simulink model "case3_primary_AGC_GFM"  (R2024b)
settings: Solver=ode15s  StartTime=0.0  StopTime=t_stop  MaxStep=0.01  RelTol=1e-6
model workspace (MATLAB code in the model file):
  | %% TWO-MACHINE SYSTEM  -  model data
  | % Case 3 - primary + secondary control (AGC) + GFM
  | % Rodriguez-Amenedo & Arnaltes Gomez, IEEE Access 9 (2021), Fig. 14.
  | % Per unit on Sbase = 100 MVA, f0 = 50 Hz, phasor (RMS) model.
  | % This code is stored in the model (Model Explorer > Model Workspace) and
  | % runs automatically when the model is opened. Edit the values here and
  | % click "Reinitialize from Source" to apply them.
  | 
  | %% Disturbance and simulation time
  | dP_L2_MW = -100;     % load step at bus 2 [MW] (paper: -100 MW, load rejection)
  | t_step   = 1;        % time of the load step [s]
  | t_stop   = 150;      % simulation time [s] (the slow AGC settles in about 125 s)
  | 
  | %% System base
  | Sbase = 100;         % [MVA]
  | f0    = 50;          % [Hz]
  | ws    = 2*pi*f0;     % [rad/s]
  | 
  | %% Network reactances [pu on 100 MVA]
  | x_T1 = 0.01;         % transformer SG1, bus 1-2
  | x_T5 = 0.01;         % transformer GFM, bus 5-2 (bus 5 = GFM connection point)
  | x_T2 = 0.003;        % transformer SG2, bus 3-4
  | x_L  = 0.2/2;        % two parallel 0.2 pu tie-lines, bus 2-3
  | 
  | %% Operating point (paper Table 2)
  | P_SG1 = 1350;                            % SG1 dispatch [MW]
  | P_L2  = 1250;  P_L3  = 4000;             % loads [MW], unity power factor
  | V1    = 1.0;   V4    = 1.0;              % [pu]; bus 4 (SG2) is the slack
  | P_GFM = 0;     Q_GFM = 0;                % GFM dispatch [MW], [MVAr]
  | 
  | %% Synchronous generators - model 0.0, classical (own rating)
  | % Constant emf E' behind the transient reactance x'd; no rotor circuits,
  | % no exciter.
  | S1  = 1500;  S2 = 4000;      % ratings [MVA]
  | H   = 6.3;                   % inertia constant [s]
  | D   = 0;                     % rotor damping [pu torque / pu speed, own base] (paper)
  | D_load = 1;                  % load damping [pu load change / pu frequency change,
  |                              % load base]: typical 1-2 (Kundur 1994, Sec. 11.1.3),
  |                              % lower end used. The paper's loads have no frequency
  |                              % dependence; the load damping is lumped into the swing
  |                              % equations as in the standard LFC model, 1/(2Hs + D).
  | D1  = D + D_load*P_L2/S1;    % total damping SG1 [pu, own base] (Area-1 load, bus 2)
  | D2  = D + D_load*P_L3/S2;    % total damping SG2 [pu, own base] (Area-2 load, bus 3)
  | xdp = 0.34;                  % transient reactance x'd [pu]
  | 
  | %% Governor and turbine - IEEEG1 (paper Table 7), primary control
  | K   = 20;                    % governor gain 1/R (5 % droop)
  | T3  = 0.1;                   % servo time constant [s]
  | Uo  = 0.5;   Uc = -0.5;      % valve rate limits [pu/s]
  | Pmax = 1;    Pmin = 0;       % valve position limits [pu]
  | T4  = 0.3;   T5 = 7;   T6 = 0.6;      % steam chest, reheater, crossover [s]
  | K1  = 0.3;   K3 = 0.3; K5 = 0.4;      % HP, IP, LP power fractions
  | 
  | kS1 = S1/Sbase;   xd1 = xdp/kS1;      % x'd of SG1 on 100 MVA
  | kS2 = S2/Sbase;   xd2 = xdp/kS2;      % x'd of SG2 on 100 MVA
  | 
  | %% Secondary control - tie-line bias AGC
  | % Area 1 = SG1 (+ GFM), Area 2 = SG2. Bias B = area frequency response
  | % (set in the AGC block). Ki: integral gain [pu set-point / pu ACE / s].
  | Ki = 0.02;     % low gain: AGC about 6-7 times slower than primary control
  | 
  | %% Grid-forming converter (own rating)
  | Sg  = 1500;                  % rating [MVA]
  | kSg = Sg/Sbase;
  | xg  = 0.15/kSg;              % coupling reactance on 100 MVA
  | Rg  = 0.05;                  % P-f droop [pu]
  | Kw  = 3;    Tw = 1;          % POD-P washout gain [pu] and time constant [s]
  | pod_on = 0;                  % 0 = pure P-f droop (POD-P washout loop off), 1 = droop + POD-P
  | Tf  = 0.02;                  % bus-frequency measurement filter [s]
  | 
  | %% Bus admittance matrix (buses 1..5)
  | Ybus     = zeros(5);
  | branches = [1 2 x_T1; 5 2 x_T5; 3 4 x_T2; 2 3 x_L];   % [from to x]
  | for k = 1:size(branches, 1)
  |     i = branches(k,1);  j = branches(k,2);  y = 1/(1i*branches(k,3));
  |     Ybus([i j], [i j]) = Ybus([i j], [i j]) + [y -y; -y y];
  | end
  | 
  | %% Load flow (Newton-Raphson)
  | % Unknowns z = [th1 th2 th3 th5 V2 V3 V5]; bus 1 PV, buses 2,3,5 PQ.
  | Vbus  = @(z) [V1*exp(1i*z(1)); z(5)*exp(1i*z(2)); z(6)*exp(1i*z(3)); V4; z(7)*exp(1i*z(4))];
  | Sinj  = @(V) V .* conj(Ybus*V);
  | PQ    = @(S) [real(S([1 2 3 5])); imag(S([2 3 5]))];
  | spec  = [P_SG1; -P_L2; -P_L3; P_GFM; 0; 0; Q_GFM] / Sbase;
  | mis   = @(z) PQ(Sinj(Vbus(z))) - spec;
  | 
  | z = [0; 0; 0; 0; 1; 1; 1];
  | for it = 1:20
  |     J = zeros(7);
  |     for k = 1:7
  |         dz = zeros(7,1);  dz(k) = 1e-7;
  |         J(:,k) = (mis(z + dz) - mis(z)) / 1e-7;
  |     end
  |     z = z - J \ mis(z);
  | end
  | if norm(mis(z)) > 1e-9
  |     error('Load flow did not converge (mismatch %.1e pu).', norm(mis(z)));
  | end
  | V0 = Vbus(z);                % bus voltages [pu]
  | S0 = Sinj(V0);               % bus injections [pu]
  | 
  | %% Initial values of the synchronous generators: E' = V + j x'd I
  | E1 = V0(1) + 1i*xd1*conj(S0(1)/V0(1));
  | E2 = V0(4) + 1i*xd2*conj(S0(4)/V0(4));
  | E1_mag = abs(E1);   delta1_0 = angle(E1);      % |E'| is held fixed
  | E2_mag = abs(E2);   delta2_0 = angle(E2);
  | Pm1_0  = real(S0(1)) / kS1;                  % governor set-points [pu own]
  | Pm2_0  = real(S0(4)) / kS2;
  | Ptie_0 = real(V0(2) * conj((V0(2) - V0(3)) / (1i*x_L)));   % scheduled tie flow [pu]
  | 
  | %% Initial values of the GFM: Eg = V + j xg I  (|Eg| is held fixed)
  | Eg = V0(5) + 1i*xg*conj(S0(5)/V0(5));
  | Eg_mag   = abs(Eg);   deltag_0 = angle(Eg);
  | Pg_ref   = real(S0(5)) / kSg;                % GFM power reference [pu own]
  | theta5_0 = angle(V0(5));
  | 
  | %% Network impedance matrices (ZI loads, as in the paper)
  | % Loads are ZI loads: the active power is a constant current in phase with
  | % the bus voltage, I_L = I_L,mag * V/|V| (so P_L is proportional to |V|);
  | % the reactive power is a constant impedance (zero here: unity power factor).
  | % The SG transient reactances x'd are added at buses 1 and 4,
  | % the GFM reactance xg at bus 5 (Norton form like the SGs).
  | % Network block: V = Zn*J - ZnL*I_L (J: Norton currents of the sources).
  | yQ      = zeros(5,1);
  | yQ(2:3) = 1i*imag(conj(-S0(2:3)) ./ abs(V0(2:3)).^2);   % constant-Z reactive part
  | Yaug    = Ybus + diag(yQ);
  | Yaug(1,1) = Yaug(1,1) + 1/(1i*xd1);
  | Yaug(4,4) = Yaug(4,4) + 1/(1i*xd2);
  | Yaug(5,5) = Yaug(5,5) + 1/(1i*xg);     % GFM reactance, Norton form like the SGs
  | Z   = inv(Yaug);
  | Zn  = Z(:, [1 4 5]);       % columns of the source (Norton) injections
  | ZnL = Z(:, [2 3]);       % columns of the load buses 2 and 3
  | 
  | % Constant-current magnitudes [pu, 100 MVA]; the load step changes the
  | % current at bus 2 by dP_L2 at nominal voltage
  | IL_pre  = real(-S0(2:3)) ./ abs(V0(2:3));
  | IL_post = IL_pre + [dP_L2_MW/Sbase/abs(V0(2)); 0];
  | 
  | % Angle of the load currents: follows the bus-voltage angle (measured
  | % relative to the SG1 rotor, so it is continuous) through a fast lag that
  | % breaks the algebraic loop through the load buses (numerical only)
  | T_L      = 1e-4;                                         % [s]
  | thetaL_0 = delta1_0 + angle(V0(2:3) * exp(-1i*delta1_0));   % [rad]
  | 
  | % Check: the network must reproduce the load flow at t = 0
  | I0  = [E1/(1i*xd1); E2/(1i*xd2); Eg/(1i*xg)];
  | IL0 = IL_pre .* V0(2:3) ./ abs(V0(2:3));
  | if max(abs(Zn*I0 - ZnL*IL0 - V0)) > 1e-9
  |     error('Network initialization does not match the load flow.');
  | end
  | clear i j k y it dz J z I0 IL0 Z Yaug yQ branches Vbus Sinj PQ spec mis E1 E2
  | clear Eg
Description:
  | Case 3 - primary + secondary control (AGC) + GFM. Two-machine load-frequency model (SG model 0.0, classical). All data in the Model Workspace; press Run.
settings Model: Creator=Hussain  LastModifiedBy=Hussain
settings DataIOCC: SaveOutput=off
settings DebuggingCC: AlgebraicLoopMsg=error

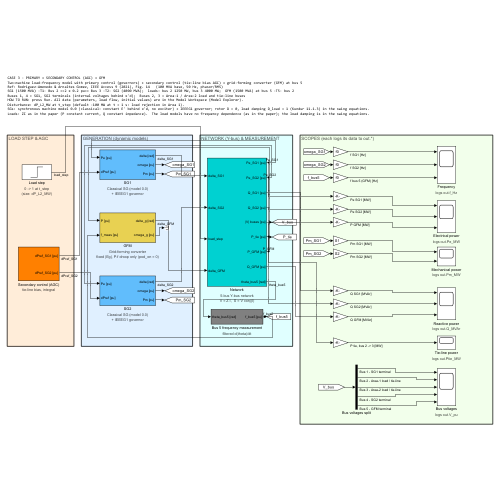
[thumbnail: Simulink's stored preview of the top-level diagram]
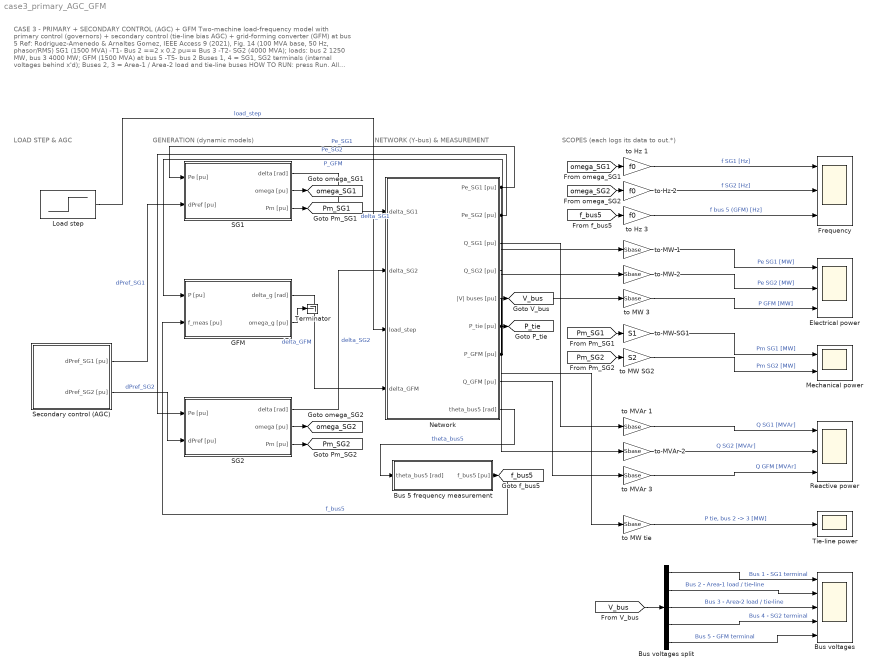
== system case3_primary_AGC_GFM ==
  note: LOAD STEP & AGC
  note: GENERATION (dynamic models)
  note: NETWORK (Y-bus) & MEASUREMENT
  note: SCOPES (each logs its data to out.*)
  note: CASE 3 - PRIMARY + SECONDARY CONTROL (AGC) + GFM
      | Two-machine load-frequency model with primary control (governors) + secondary control (tie-line bias AGC) + grid-forming converter (GFM) at bus 5
      | Ref: Rodriguez-Amenedo & Arnaltes Gomez, IEEE Access 9 (2021), Fig. 14   (100 MVA base, 50 Hz, phasor/RMS)
      | SG1 (1500 MVA) -T1- Bus 2 ==2 x 0.2 pu== Bus 3 -T2- SG2 (4000 MVA);  loads: bus 2 1250 MW, bus 3 4000 MW;  GFM (1500 MVA) at bus 5 -T5- bus 2
      | Buses 1, 4 = SG1, SG2 terminals (internal voltages behind x'd);  Buses 2, 3 = Area-1 / Area-2 load and tie-line buses
      | HOW TO RUN: press Run. All data (parameters, load flow, initial values) are in the Model Workspace (Model Explorer).
      | Disturbance: dP_L2_MW at t_step (default -100 MW at t = 1 s: load rejection in Area 1).
      | SGs: synchronous machine model 0.0 (classical: constant E' behind x'd, no exciter) + IEEEG1 governor; rotor D = 0, load damping D_load = 1 (Kundur 11.1.3) in the swing equations.
      | Loads: ZI as in the paper (P constant current, Q constant impedance).  The load models have no frequency dependence (as in the paper); the load damping is in the swing equations.
  Bus 5 frequency measurement : Subsystem
      settings: AttributesFormatString=filtered d(theta)/dt
  Bus voltages : Scope  NumInputPorts=5
      settings: AttributesFormatString=logs out.V_pu
  Bus voltages split : Demux  Outputs=5
  Electrical power : Scope  NumInputPorts=3
      settings: AttributesFormatString=logs out.Pe_MW
  Frequency : Scope  NumInputPorts=3
      settings: AttributesFormatString=logs out.f_Hz
  GFM : Subsystem
      settings: AttributesFormatString=Grid-forming converter\nfixed |Eg|, P-f droop only (pod_on = 0)
  Load step : Step  Time=t_step  SampleTime=0
      settings: AttributesFormatString=0 -> 1 at t_step\n(size: dP_L2_MW)
  Mechanical power : Scope  NumInputPorts=2
      settings: AttributesFormatString=logs out.Pm_MW
  Network : Subsystem
      settings: AttributesFormatString="5-bus Y-bus network\\nV = Z I,  S = V conj(I)"
  Reactive power : Scope  NumInputPorts=3
      settings: AttributesFormatString=logs out.Q_MVAr
  SG1 : Subsystem
      settings: AttributesFormatString=Classical SG (model 0.0)\n+ IEEEG1 governor
  SG2 : Subsystem
      settings: AttributesFormatString=Classical SG (model 0.0)\n+ IEEEG1 governor
  Secondary control (AGC) : Subsystem
      settings: AttributesFormatString=tie-line bias, integral
  Terminator : Terminator
  Tie-line power : Scope
      settings: AttributesFormatString=logs out.Ptie_MW
  to Hz 1 : Gain  Gain=f0
  to Hz 2 : Gain  Gain=f0
  to Hz 3 : Gain  Gain=f0
  to MVAr 1 : Gain  Gain=Sbase
  to MVAr 2 : Gain  Gain=Sbase
  to MVAr 3 : Gain  Gain=Sbase
  to MW 1 : Gain  Gain=Sbase
  to MW 2 : Gain  Gain=Sbase
  to MW 3 : Gain  Gain=Sbase
  to MW SG1 : Gain  Gain=S1
  to MW SG2 : Gain  Gain=S2
  to MW tie : Gain  Gain=Sbase
  tag scope: P_tie=global, Pm_SG1=global, Pm_SG2=global, V_bus=global, f_bus5=global, omega_SG1=global, omega_SG2=global
  wires:
  Secondary control (AGC)/1(dPref_SG1 [pu]) -> SG1/2(dPref [pu])  "dPref_SG1"
  Secondary control (AGC)/2(dPref_SG2 [pu]) -> SG2/2(dPref [pu])  "dPref_SG2"
  SG1/1(delta [rad]) -> Network/1(delta_SG1)  "delta_SG1"
  SG2/1(delta [rad]) -> Network/2(delta_SG2)  "delta_SG2"
  Load step/1 -> Network/3(load_step)  "load_step"
  Network/1(Pe_SG1 [pu]) -> SG1/1(Pe [pu]), to MW 1/1  "Pe_SG1"
  Network/2(Pe_SG2 [pu]) -> SG2/1(Pe [pu]), to MW 2/1  "Pe_SG2"
  SG1/2(omega [pu]) -> [omega_SG1]
  SG1/3(Pm [pu]) -> [Pm_SG1]
  SG2/2(omega [pu]) -> [omega_SG2]
  SG2/3(Pm [pu]) -> [Pm_SG2]
  Network/6(P_tie [pu]) -> [P_tie], to MW tie/1
  GFM/1(delta_g [rad]) -> Network/4(delta_GFM)  "delta_GFM"
  Network/7(P_GFM [pu]) -> GFM/1(P [pu]), to MW 3/1  "P_GFM"
  Network/9(theta_bus5 [rad]) -> Bus 5 frequency measurement/1(theta_bus5 [rad])  "theta_bus5"
  Bus 5 frequency measurement/1(f_bus5 [pu]) -> GFM/2(f_meas [pu]), [f_bus5]  "f_bus5"
  GFM/2(omega_g [pu]) -> Terminator/1
  [omega_SG1] -> to Hz 1/1
  [omega_SG2] -> to Hz 2/1
  [f_bus5] -> to Hz 3/1
  to Hz 1/1 -> Frequency/1  "f SG1 [Hz]"
  to Hz 2/1 -> Frequency/2  "f SG2 [Hz]"
  to Hz 3/1 -> Frequency/3  "f bus 5 (GFM) [Hz]"
  to MW 1/1 -> Electrical power/1  "Pe SG1 [MW]"
  to MW 2/1 -> Electrical power/2  "Pe SG2 [MW]"
  to MW 3/1 -> Electrical power/3  "P GFM [MW]"
  [Pm_SG1] -> to MW SG1/1
  [Pm_SG2] -> to MW SG2/1
  to MW SG1/1 -> Mechanical power/1  "Pm SG1 [MW]"
  to MW SG2/1 -> Mechanical power/2  "Pm SG2 [MW]"
  Network/3(Q_SG1 [pu]) -> to MVAr 1/1
  Network/4(Q_SG2 [pu]) -> to MVAr 2/1
  Network/8(Q_GFM [pu]) -> to MVAr 3/1
  to MVAr 1/1 -> Reactive power/1  "Q SG1 [MVAr]"
  to MVAr 2/1 -> Reactive power/2  "Q SG2 [MVAr]"
  to MVAr 3/1 -> Reactive power/3  "Q GFM [MVAr]"
  to MW tie/1 -> Tie-line power/1  "P tie, bus 2 -> 3 [MW]"
  Network/5(|V| buses [pu]) -> [V_bus]
  [V_bus] -> Bus voltages split/1
  Bus voltages split/1 -> Bus voltages/1  "Bus 1 - SG1 terminal"
  Bus voltages split/2 -> Bus voltages/2  "Bus 2 - Area-1 load / tie-line"
  Bus voltages split/3 -> Bus voltages/3  "Bus 3 - Area-2 load / tie-line"
  Bus voltages split/4 -> Bus voltages/4  "Bus 4 - SG2 terminal"
  Bus voltages split/5 -> Bus voltages/5  "Bus 5 - GFM terminal"

== system case3_primary_AGC_GFM/Bus 5 frequency measurement ==
  note: BUS FREQUENCY MEASUREMENT (bus 5, GFM terminal)
      | Tf dx/dt = theta - x,    f = 1 + (theta - x) / (Tf omega_s)   [pu]
      | A first-order filtered derivative of the bus voltage angle.
  theta_bus5 [rad] : Inport
  Angle error : Sum  Inputs=+-
  Bus frequency : Sum
  Filtered angle : Integrator  InitialCondition=theta5_0
  Nominal 1 pu : Constant
  One over Tf : Gain  Gain=1/Tf
  to pu frequency : Gain  Gain=1/ws
  f_bus5 [pu] : Outport
  wires:
  One over Tf/1 -> Filtered angle/1, to pu frequency/1  "d(theta)/dt"
  Bus frequency/1 -> f_bus5 [pu]/1  "f_bus5"
  to pu frequency/1 -> Bus frequency/2
  Nominal 1 pu/1 -> Bus frequency/1
  Angle error/1 -> One over Tf/1
  theta_bus5 [rad]/1 -> Angle error/1
  Filtered angle/1 -> Angle error/2

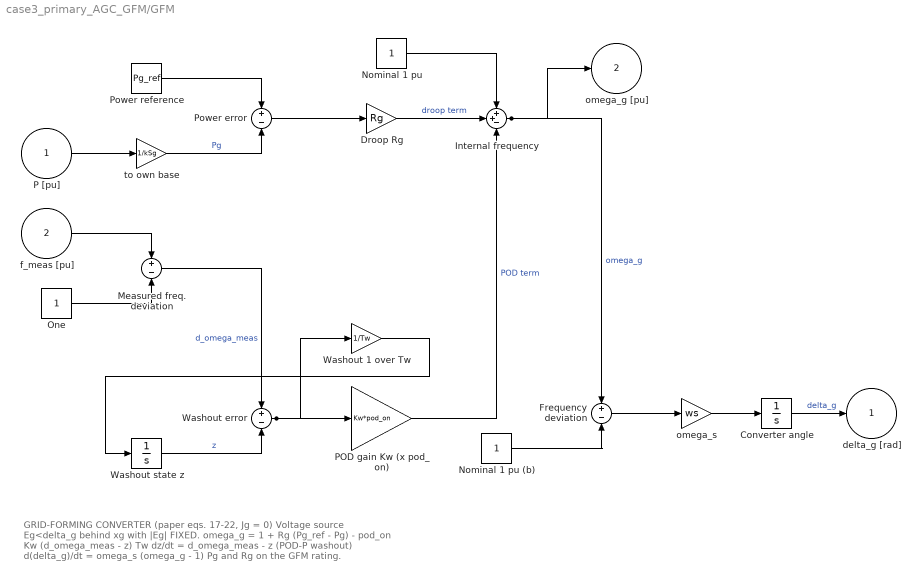
== system case3_primary_AGC_GFM/GFM ==
  note: GRID-FORMING CONVERTER (paper eqs. 17-22, Jg = 0)
      | Voltage source Eg<delta_g behind xg with |Eg| FIXED.
      | omega_g = 1 + Rg (Pg_ref - Pg) - pod_on Kw (d_omega_meas - z)
      | Tw dz/dt = d_omega_meas - z          (POD-P washout)
      | d(delta_g)/dt = omega_s (omega_g - 1)
      | Pg and Rg on the GFM rating.
  P [pu] : Inport
  f_meas [pu] : Inport  Port=2
  Converter angle : Integrator  InitialCondition=deltag_0
  Droop Rg : Gain  Gain=Rg
  Frequency deviation : Sum  Inputs=+-
  Internal frequency : Sum  Inputs=++-
  Measured freq. deviation : Sum  Inputs=+-
  Nominal 1 pu : Constant
  Nominal 1 pu (b) : Constant
  One : Constant
  POD gain Kw (x pod_on) : Gain  Gain=Kw*pod_on
  Power error : Sum  Inputs=+-
  Power reference : Constant  Value=Pg_ref
  Washout 1 over Tw : Gain  Gain=1/Tw
  Washout error : Sum  Inputs=+-
  Washout state z : Integrator
  omega_s : Gain  Gain=ws
  to own base : Gain  Gain=1/kSg
  delta_g [rad] : Outport
  omega_g [pu] : Outport  Port=2
  wires:
  P [pu]/1 -> to own base/1
  f_meas [pu]/1 -> Measured freq. deviation/1
  Converter angle/1 -> delta_g [rad]/1  "delta_g"
  Measured freq. deviation/1 -> Washout error/1  "d_omega_meas"
  One/1 -> Measured freq. deviation/2
  Power error/1 -> Droop Rg/1
  Power reference/1 -> Power error/1
  Washout state z/1 -> Washout error/2  "z"
  to own base/1 -> Power error/2  "Pg"
  Washout error/1 -> POD gain Kw (x pod_on)/1, Washout 1 over Tw/1
  Nominal 1 pu/1 -> Internal frequency/1
  Frequency deviation/1 -> omega_s/1
  Droop Rg/1 -> Internal frequency/2  "droop term"
  Washout 1 over Tw/1 -> Washout state z/1
  POD gain Kw (x pod_on)/1 -> Internal frequency/3  "POD term"
  Internal frequency/1 -> Frequency deviation/1, omega_g [pu]/1  "omega_g"
  Nominal 1 pu (b)/1 -> Frequency deviation/2
  omega_s/1 -> Converter angle/1

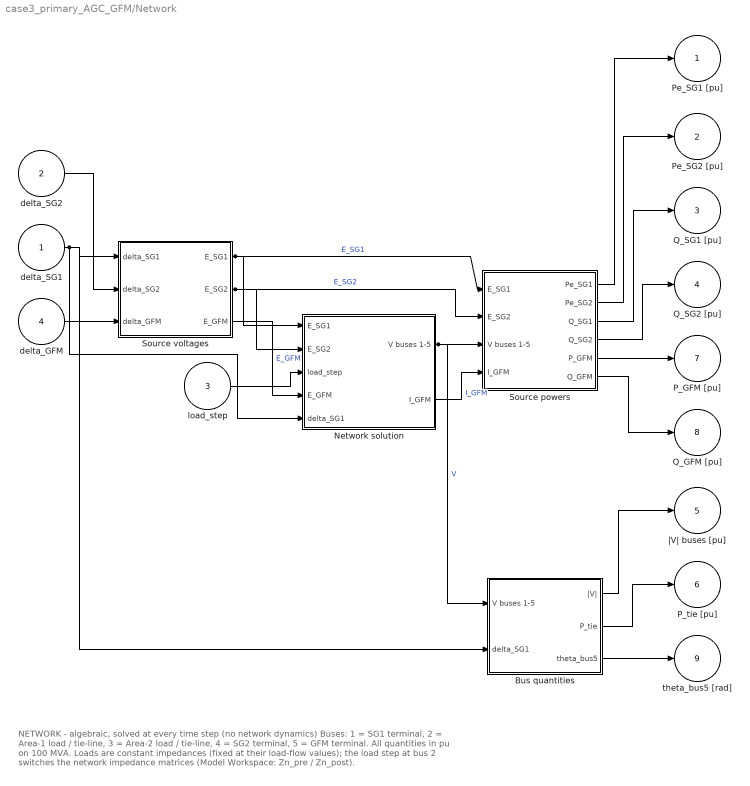
== system case3_primary_AGC_GFM/Network ==
  note: NETWORK - algebraic, solved at every time step (no network dynamics)
      | Buses: 1 = SG1 terminal, 2 = Area-1 load / tie-line, 3 = Area-2 load / tie-line,
      |        4 = SG2 terminal, 5 = GFM terminal.  All quantities in pu on 100 MVA.
      | Loads are constant impedances (fixed at their load-flow values); the load step at
      | bus 2 switches the network impedance matrices (Model Workspace: Zn_pre / Zn_post).
  delta_SG1 : Inport
  delta_SG2 : Inport  Port=2
  load_step : Inport  Port=3
  delta_GFM : Inport  Port=4
  Bus quantities : Subsystem
      settings: AttributesFormatString=|V|, tie-line flow, bus-5 angle
  Network solution : Subsystem
      settings: AttributesFormatString=V = Zn [J_SG1; J_SG2; J_GFM]
  Source powers : Subsystem
      settings: AttributesFormatString=S = V_terminal conj(I)
  Source voltages : Subsystem
      settings: AttributesFormatString=E = |E| at angle delta
  Pe_SG1 [pu] : Outport
  Pe_SG2 [pu] : Outport  Port=2
  Q_SG1 [pu] : Outport  Port=3
  Q_SG2 [pu] : Outport  Port=4
  |V| buses [pu] : Outport  Port=5
  P_tie [pu] : Outport  Port=6
  P_GFM [pu] : Outport  Port=7
  Q_GFM [pu] : Outport  Port=8
  theta_bus5 [rad] : Outport  Port=9
  wires:
  delta_SG2/1 -> Source voltages/2(delta_SG2)
  load_step/1 -> Network solution/3(load_step)
  delta_SG1/1 -> Bus quantities/2(delta_SG1), Source voltages/1(delta_SG1), Network solution/5(delta_SG1)
  Network solution/1(V buses 1-5) -> Source powers/3(V buses 1-5), Bus quantities/1(V buses 1-5)  "V"
  delta_GFM/1 -> Source voltages/3(delta_GFM)
  Source voltages/1(E_SG1) -> Source powers/1(E_SG1), Network solution/1(E_SG1)  "E_SG1"
  Source voltages/3(E_GFM) -> Network solution/4(E_GFM)  "E_GFM"
  Source voltages/2(E_SG2) -> Source powers/2(E_SG2), Network solution/2(E_SG2)  "E_SG2"
  Network solution/2(I_GFM) -> Source powers/4(I_GFM)  "I_GFM"
  Source powers/1(Pe_SG1) -> Pe_SG1 [pu]/1
  Source powers/2(Pe_SG2) -> Pe_SG2 [pu]/1
  Source powers/3(Q_SG1) -> Q_SG1 [pu]/1
  Source powers/4(Q_SG2) -> Q_SG2 [pu]/1
  Source powers/5(P_GFM) -> P_GFM [pu]/1
  Source powers/6(Q_GFM) -> Q_GFM [pu]/1
  Bus quantities/1(|V|) -> |V| buses [pu]/1
  Bus quantities/2(P_tie) -> P_tie [pu]/1
  Bus quantities/3(theta_bus5) -> theta_bus5 [rad]/1

== system case3_primary_AGC_GFM/SG1 ==
  note: SG1 - SYNCHRONOUS GENERATOR, MODEL 0.0 (classical)
      | Constant emf E'1 behind x'd (no rotor circuits, no exciter). The network returns Pe;
      | the swing equation gives speed and rotor angle; governor + turbine set Pm.
  Pe [pu] : Inport
  dPref [pu] : Inport  Port=2
  Governor (IEEEG1) : Subsystem
  Swing equation : Subsystem
  Turbine (reheat) : Subsystem
  delta [rad] : Outport
  omega [pu] : Outport  Port=2
  Pm [pu] : Outport  Port=3
  wires:
  Turbine (reheat)/1(Pm [pu]) -> Swing equation/1(Pm [pu own]), Pm [pu]/1  "Pm"
  Pe [pu]/1 -> Swing equation/2(Pe [pu 100 MVA])  "Pe"
  Swing equation/1(delta [rad]) -> delta [rad]/1  "delta"
  dPref [pu]/1 -> Governor (IEEEG1)/2(dPref (AGC) [pu])  "dPref"
  Governor (IEEEG1)/1(valve gv [pu]) -> Turbine (reheat)/1(valve gv [pu])  "gv"
  Swing equation/2(omega [pu]) -> Governor (IEEEG1)/1(omega [pu]), omega [pu]/1  "omega"

== system case3_primary_AGC_GFM/SG2 ==
  note: SG2 - SYNCHRONOUS GENERATOR, MODEL 0.0 (classical)
      | Constant emf E'2 behind x'd (no rotor circuits, no exciter). The network returns Pe;
      | the swing equation gives speed and rotor angle; governor + turbine set Pm.
  Pe [pu] : Inport
  dPref [pu] : Inport  Port=2
  Governor (IEEEG1) : Subsystem
  Swing equation : Subsystem
  Turbine (reheat) : Subsystem
  delta [rad] : Outport
  omega [pu] : Outport  Port=2
  Pm [pu] : Outport  Port=3
  wires:
  Turbine (reheat)/1(Pm [pu]) -> Swing equation/1(Pm [pu own]), Pm [pu]/1  "Pm"
  Pe [pu]/1 -> Swing equation/2(Pe [pu 100 MVA])  "Pe"
  dPref [pu]/1 -> Governor (IEEEG1)/2(dPref (AGC) [pu])  "dPref"
  Swing equation/1(delta [rad]) -> delta [rad]/1  "delta"
  Governor (IEEEG1)/1(valve gv [pu]) -> Turbine (reheat)/1(valve gv [pu])  "gv"
  Swing equation/2(omega [pu]) -> Governor (IEEEG1)/1(omega [pu]), omega [pu]/1  "omega"

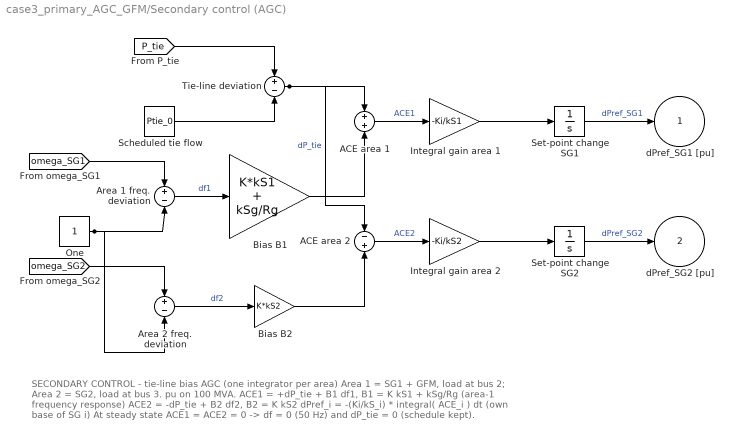
== system case3_primary_AGC_GFM/Secondary control (AGC) ==
  note: SECONDARY CONTROL - tie-line bias AGC (one integrator per area)
      | Area 1 = SG1 + GFM, load at bus 2;  Area 2 = SG2, load at bus 3.  pu on 100 MVA.
      | ACE1 = +dP_tie + B1 df1,   B1 = K kS1 + kSg/Rg   (area-1 frequency response)
      | ACE2 = -dP_tie + B2 df2,   B2 = K kS2
      | dPref_i = -(Ki/kS_i) * integral( ACE_i ) dt      (own base of SG i)
      | At steady state ACE1 = ACE2 = 0  ->  df = 0 (50 Hz) and dP_tie = 0 (schedule kept).
  ACE area 1 : Sum
  ACE area 2 : Sum  Inputs=-+
  Area 1 freq. deviation : Sum  Inputs=+-
  Area 2 freq. deviation : Sum  Inputs=+-
  Bias B1 : Gain  Gain=K*kS1 + kSg/Rg
  Bias B2 : Gain  Gain=K*kS2
  Integral gain area 1 : Gain  Gain=-Ki/kS1
  Integral gain area 2 : Gain  Gain=-Ki/kS2
  One : Constant
  Scheduled tie flow : Constant  Value=Ptie_0
  Set-point change SG1 : Integrator
  Set-point change SG2 : Integrator
  Tie-line deviation : Sum  Inputs=+-
  dPref_SG1 [pu] : Outport
  dPref_SG2 [pu] : Outport  Port=2
  wires:
  [omega_SG1] -> Area 1 freq. deviation/1
  Tie-line deviation/1 -> ACE area 2/1, ACE area 1/1  "dP_tie"
  Area 2 freq. deviation/1 -> Bias B2/1  "df2"
  Integral gain area 2/1 -> Set-point change SG2/1
  Area 1 freq. deviation/1 -> Bias B1/1  "df1"
  One/1 -> Area 2 freq. deviation/2, Area 1 freq. deviation/2
  [omega_SG2] -> Area 2 freq. deviation/1
  Scheduled tie flow/1 -> Tie-line deviation/2
  Bias B2/1 -> ACE area 2/2
  [P_tie] -> Tie-line deviation/1
  Bias B1/1 -> ACE area 1/2
  ACE area 1/1 -> Integral gain area 1/1  "ACE1"
  ACE area 2/1 -> Integral gain area 2/1  "ACE2"
  Integral gain area 1/1 -> Set-point change SG1/1
  Set-point change SG1/1 -> dPref_SG1 [pu]/1  "dPref_SG1"
  Set-point change SG2/1 -> dPref_SG2 [pu]/1  "dPref_SG2"

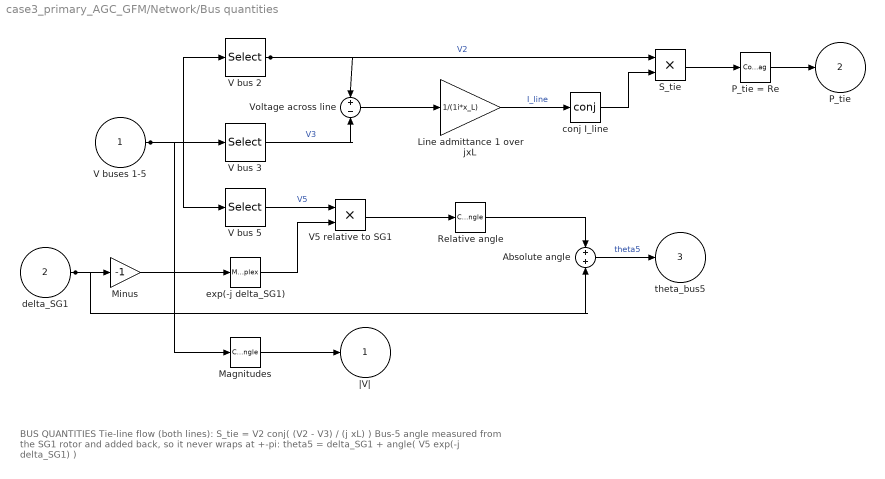
== system case3_primary_AGC_GFM/Network/Bus quantities ==
  note: BUS QUANTITIES
      | Tie-line flow (both lines): S_tie = V2 conj( (V2 - V3) / (j xL) )
      | Bus-5 angle measured from the SG1 rotor and added back, so it never wraps at +-pi:
      | theta5 = delta_SG1 + angle( V5 exp(-j delta_SG1) )
  V buses 1-5 : Inport
  delta_SG1 : Inport  Port=2
  Absolute angle : Sum
  Line admittance 1 over jxL : Gain  Gain=1/(1i*x_L)
  Magnitudes : ComplexToMagnitudeAngle  Output=Magnitude
  Minus : Gain  Gain=-1
  P_tie = Re : ComplexToRealImag  Output=Real
  Relative angle : ComplexToMagnitudeAngle  Output=Angle
  S_tie : Product
  V bus 2 : Selector  InputPortWidth=5  IndexOptions=Index vector (dialog)  Indices=2  OutputSizes=1
  V bus 3 : Selector  InputPortWidth=5  IndexOptions=Index vector (dialog)  Indices=3  OutputSizes=1
  V bus 5 : Selector  InputPortWidth=5  IndexOptions=Index vector (dialog)  Indices=5  OutputSizes=1
  V5 relative to SG1 : Product
  Voltage across line : Sum  Inputs=+-
  conj I_line : Math  Operator=conj
  exp(-j delta_SG1) : MagnitudeAngleToComplex  Input=Angle  ConstantPart=1
  |V| : Outport
  P_tie : Outport  Port=2
  theta_bus5 : Outport  Port=3
  wires:
  V buses 1-5/1 -> V bus 2/1, V bus 5/1, V bus 3/1, Magnitudes/1
  P_tie = Re/1 -> P_tie/1
  delta_SG1/1 -> Absolute angle/2, Minus/1
  exp(-j delta_SG1)/1 -> V5 relative to SG1/2
  Minus/1 -> exp(-j delta_SG1)/1
  V bus 2/1 -> Voltage across line/1, S_tie/1  "V2"
  Magnitudes/1 -> |V|/1
  V bus 3/1 -> Voltage across line/2  "V3"
  V bus 5/1 -> V5 relative to SG1/1  "V5"
  Voltage across line/1 -> Line admittance 1 over jxL/1
  V5 relative to SG1/1 -> Relative angle/1
  Line admittance 1 over jxL/1 -> conj I_line/1  "I_line"
  Relative angle/1 -> Absolute angle/1
  conj I_line/1 -> S_tie/2
  Absolute angle/1 -> theta_bus5/1  "theta5"
  S_tie/1 -> P_tie = Re/1

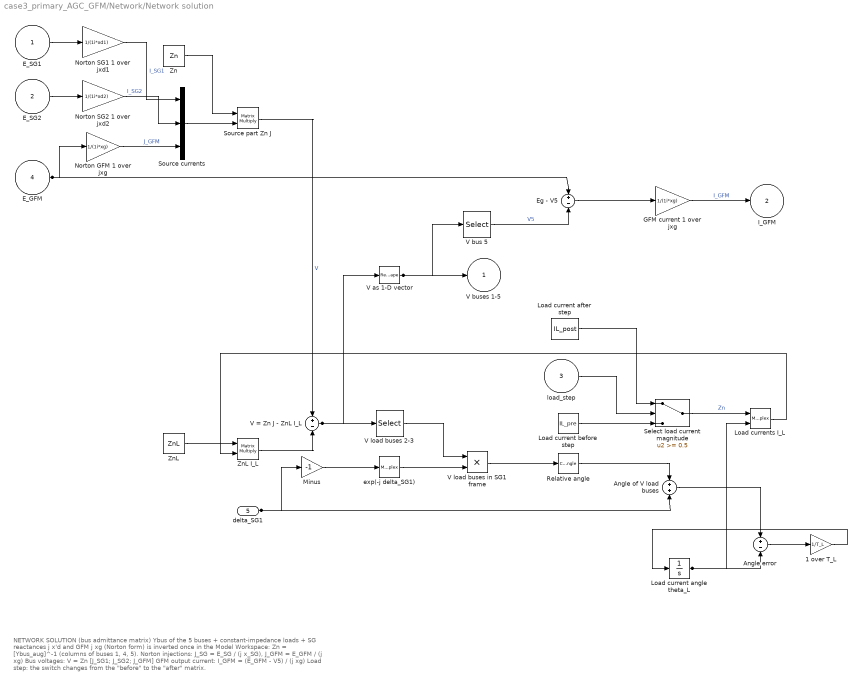
== system case3_primary_AGC_GFM/Network/Network solution ==
  note: NETWORK SOLUTION (bus admittance matrix)
      | Ybus of the 5 buses + constant-impedance loads + SG reactances j x'd and GFM j xg (Norton form)
      | is inverted once in the Model Workspace:  Zn = [Ybus_aug]^-1 (columns of buses 1, 4, 5).
      | Norton injections:  J_SG = E_SG / (j x_SG),   J_GFM = E_GFM / (j xg)
      | Bus voltages:       V = Zn [J_SG1; J_SG2; J_GFM]
      | GFM output current: I_GFM = (E_GFM - V5) / (j xg)
      | Load step: the switch changes from the "before" to the "after" matrix.
  E_SG1 : Inport
  E_SG2 : Inport  Port=2
  load_step : Inport  Port=3
  E_GFM : Inport  Port=4
  delta_SG1 : Inport  Port=5
  1 over T_L : Gain  Gain=1/T_L
  Angle error : Sum  Inputs=+-
  Angle of V load buses : Sum
  Eg - V5 : Sum  Inputs=+-
  GFM current 1 over jxg : Gain  Gain=1/(1i*xg)
  Load current after step : Constant  Value=IL_post  VectorParams1D=off
  Load current angle theta_L : Integrator  InitialCondition=thetaL_0
  Load current before step : Constant  Value=IL_pre  VectorParams1D=off
  Load currents I_L : MagnitudeAngleToComplex
  Minus : Gain  Gain=-1
  Norton GFM 1 over jxg : Gain  Gain=1/(1i*xg)
  Norton SG1 1 over jxd1 : Gain  Gain=1/(1i*xd1)
  Norton SG2 1 over jxd2 : Gain  Gain=1/(1i*xd2)
  Relative angle : ComplexToMagnitudeAngle  Output=Angle
  Select load current magnitude : Switch  Threshold=0.5  SaturateOnIntegerOverflow=off  InputSameDT=off
  Source currents : Mux  Inputs=3
  Source part Zn J : Product  Multiplication=Matrix(*)
  V = Zn J - ZnL I_L : Sum  Inputs=+-
  V as 1-D vector : Reshape
  V bus 5 : Selector  InputPortWidth=5  IndexOptions=Index vector (dialog)  Indices=5  OutputSizes=1
  V load buses 2-3 : Selector  InputPortWidth=5  IndexOptions=Index vector (dialog)  Indices=[2 3]  OutputSizes=1
  V load buses in SG1 frame : Product  Inputs=**
  Zn : Constant  Value=Zn
  ZnL : Constant  Value=ZnL
  ZnL I_L : Product  Inputs=**  Multiplication=Matrix(*)
  exp(-j delta_SG1) : MagnitudeAngleToComplex  Input=Angle  ConstantPart=1
  V buses 1-5 : Outport
  I_GFM : Outport  Port=2
  wires:
  E_SG1/1 -> Norton SG1 1 over jxd1/1
  E_GFM/1 -> Eg - V5/1, Norton GFM 1 over jxg/1
  E_SG2/1 -> Norton SG2 1 over jxd2/1
  Norton GFM 1 over jxg/1 -> Source currents/3  "J_GFM"
  Norton SG1 1 over jxd1/1 -> Source currents/1  "I_SG1"
  V load buses 2-3/1 -> V load buses in SG1 frame/1
  Source part Zn J/1 -> V = Zn J - ZnL I_L/1  "V"
  Norton SG2 1 over jxd2/1 -> Source currents/2  "I_SG2"
  Zn/1 -> Source part Zn J/1
  Source currents/1 -> Source part Zn J/2
  Relative angle/1 -> Angle of V load buses/1
  ZnL/1 -> ZnL I_L/1
  ZnL I_L/1 -> V = Zn J - ZnL I_L/2
  exp(-j delta_SG1)/1 -> V load buses in SG1 frame/2
  delta_SG1/1 -> Angle of V load buses/2, Minus/1
  Minus/1 -> exp(-j delta_SG1)/1
  V = Zn J - ZnL I_L/1 -> V as 1-D vector/1, V load buses 2-3/1
  V as 1-D vector/1 -> V buses 1-5/1, V bus 5/1
  V bus 5/1 -> Eg - V5/2  "V5"
  V load buses in SG1 frame/1 -> Relative angle/1
  Eg - V5/1 -> GFM current 1 over jxg/1
  Load current after step/1 -> Select load current magnitude/1
  load_step/1 -> Select load current magnitude/2
  Load current before step/1 -> Select load current magnitude/3
  GFM current 1 over jxg/1 -> I_GFM/1  "I_GFM"
  Angle error/1 -> 1 over T_L/1
  Select load current magnitude/1 -> Load currents I_L/1  "Zn"
  Angle of V load buses/1 -> Angle error/1
  Load current angle theta_L/1 -> Angle error/2, Load currents I_L/2
  Load currents I_L/1 -> ZnL I_L/2
  1 over T_L/1 -> Load current angle theta_L/1

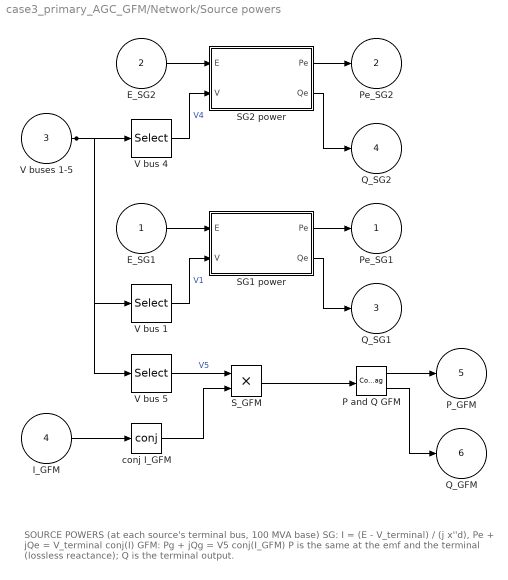
== system case3_primary_AGC_GFM/Network/Source powers ==
  note: SOURCE POWERS (at each source's terminal bus, 100 MVA base)
      | SG:  I = (E - V_terminal) / (j x''d),   Pe + jQe = V_terminal conj(I)
      | GFM: Pg + jQg = V5 conj(I_GFM)
      | P is the same at the emf and the terminal (lossless reactance); Q is the terminal output.
  E_SG1 : Inport
  E_SG2 : Inport  Port=2
  V buses 1-5 : Inport  Port=3
  I_GFM : Inport  Port=4
  P and Q GFM : ComplexToRealImag
  SG1 power : Subsystem
      settings: AttributesFormatString="S = V conj(I);  I = (E-V)/(j xd1)"
  SG2 power : Subsystem
      settings: AttributesFormatString="S = V conj(I);  I = (E-V)/(j xd2)"
  S_GFM : Product
  V bus 1 : Selector  InputPortWidth=5  IndexOptions=Index vector (dialog)  Indices=1  OutputSizes=1
  V bus 4 : Selector  InputPortWidth=5  IndexOptions=Index vector (dialog)  Indices=4  OutputSizes=1
  V bus 5 : Selector  InputPortWidth=5  IndexOptions=Index vector (dialog)  Indices=5  OutputSizes=1
  conj I_GFM : Math  Operator=conj
  Pe_SG1 : Outport
  Pe_SG2 : Outport  Port=2
  Q_SG1 : Outport  Port=3
  Q_SG2 : Outport  Port=4
  P_GFM : Outport  Port=5
  Q_GFM : Outport  Port=6
  wires:
  I_GFM/1 -> conj I_GFM/1
  V buses 1-5/1 -> V bus 1/1, V bus 4/1, V bus 5/1
  E_SG2/1 -> SG2 power/1(E)
  V bus 4/1 -> SG2 power/2(V)  "V4"
  V bus 5/1 -> S_GFM/1  "V5"
  E_SG1/1 -> SG1 power/1(E)
  V bus 1/1 -> SG1 power/2(V)  "V1"
  conj I_GFM/1 -> S_GFM/2
  SG2 power/1(Pe) -> Pe_SG2/1
  SG2 power/2(Qe) -> Q_SG2/1
  SG1 power/1(Pe) -> Pe_SG1/1
  SG1 power/2(Qe) -> Q_SG1/1
  S_GFM/1 -> P and Q GFM/1
  P and Q GFM/1 -> P_GFM/1
  P and Q GFM/2 -> Q_GFM/1

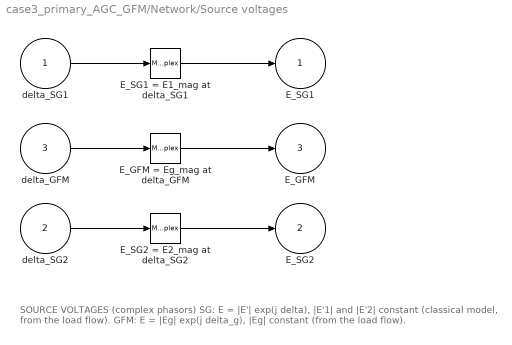
== system case3_primary_AGC_GFM/Network/Source voltages ==
  note: SOURCE VOLTAGES (complex phasors)
      | SG: E = |E'| exp(j delta), |E'1| and |E'2| constant (classical model, from the load flow).
      | GFM: E = |Eg| exp(j delta_g), |Eg| constant (from the load flow).
  delta_SG1 : Inport
  delta_SG2 : Inport  Port=2
  delta_GFM : Inport  Port=3
  E_GFM = Eg_mag at delta_GFM : MagnitudeAngleToComplex  Input=Angle  ConstantPart=Eg_mag
  E_SG1 = E1_mag at delta_SG1 : MagnitudeAngleToComplex  Input=Angle  ConstantPart=E1_mag
  E_SG2 = E2_mag at delta_SG2 : MagnitudeAngleToComplex  Input=Angle  ConstantPart=E2_mag
  E_SG1 : Outport
  E_SG2 : Outport  Port=2
  E_GFM : Outport  Port=3
  wires:
  delta_SG1/1 -> E_SG1 = E1_mag at delta_SG1/1
  E_GFM = Eg_mag at delta_GFM/1 -> E_GFM/1
  E_SG1 = E1_mag at delta_SG1/1 -> E_SG1/1
  delta_GFM/1 -> E_GFM = Eg_mag at delta_GFM/1
  delta_SG2/1 -> E_SG2 = E2_mag at delta_SG2/1
  E_SG2 = E2_mag at delta_SG2/1 -> E_SG2/1

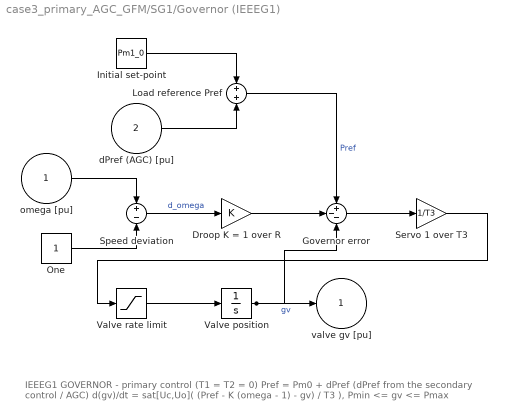
== system case3_primary_AGC_GFM/SG1/Governor (IEEEG1) ==
  note: IEEEG1 GOVERNOR - primary control (T1 = T2 = 0)
      | Pref = Pm0 + dPref   (dPref from the secondary control / AGC)
      | d(gv)/dt = sat[Uc,Uo]( (Pref - K (omega - 1) - gv) / T3 ),  Pmin <= gv <= Pmax
  omega [pu] : Inport
  dPref (AGC) [pu] : Inport  Port=2
  Droop K = 1 over R : Gain  Gain=K
  Governor error : Sum  Inputs=+--
  Initial set-point : Constant  Value=Pm1_0
  Load reference Pref : Sum
  One : Constant
  Servo 1 over T3 : Gain  Gain=1/T3
  Speed deviation : Sum  Inputs=+-
  Valve position : Integrator  InitialCondition=Pm1_0  LimitOutput=on  UpperSaturationLimit=Pmax  LowerSaturationLimit=Pmin
  Valve rate limit : Saturate  UpperLimit=Uo  LowerLimit=Uc
  valve gv [pu] : Outport
  wires:
  Droop K = 1 over R/1 -> Governor error/2
  omega [pu]/1 -> Speed deviation/1
  Load reference Pref/1 -> Governor error/1  "Pref"
  Speed deviation/1 -> Droop K = 1 over R/1  "d_omega"
  Initial set-point/1 -> Load reference Pref/1
  One/1 -> Speed deviation/2
  dPref (AGC) [pu]/1 -> Load reference Pref/2
  Valve rate limit/1 -> Valve position/1
  Valve position/1 -> Governor error/3, valve gv [pu]/1  "gv"
  Governor error/1 -> Servo 1 over T3/1
  Servo 1 over T3/1 -> Valve rate limit/1

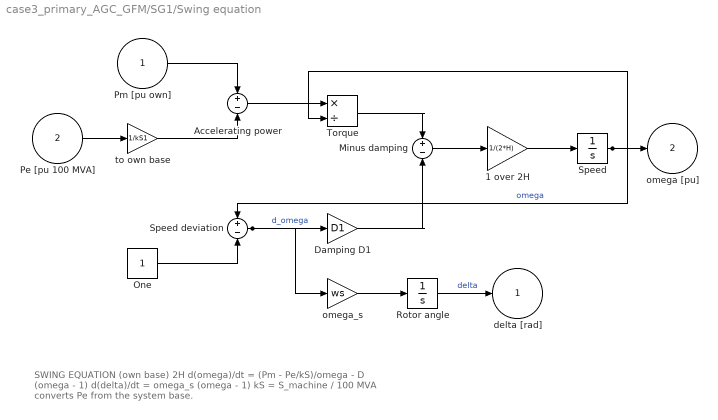
== system case3_primary_AGC_GFM/SG1/Swing equation ==
  note: SWING EQUATION (own base)
      | 2H d(omega)/dt = (Pm - Pe/kS)/omega - D (omega - 1)
      | d(delta)/dt    = omega_s (omega - 1)
      | kS = S_machine / 100 MVA converts Pe from the system base.
  Pm [pu own] : Inport
  Pe [pu 100 MVA] : Inport  Port=2
  1 over 2H : Gain  Gain=1/(2*H)
  Accelerating power : Sum  Inputs=+-
  Damping D1 : Gain  Gain=D1
  Minus damping : Sum  Inputs=+-
  One : Constant
  Rotor angle : Integrator  InitialCondition=delta1_0
  Speed : Integrator  InitialCondition=1
  Speed deviation : Sum  Inputs=+-
  Torque : Product  Inputs=*/
  omega_s : Gain  Gain=ws
  to own base : Gain  Gain=1/kS1
  delta [rad] : Outport
  omega [pu] : Outport  Port=2
  wires:
  Pe [pu 100 MVA]/1 -> to own base/1
  Damping D1/1 -> Minus damping/2
  Pm [pu own]/1 -> Accelerating power/1
  Torque/1 -> Minus damping/1
  Speed deviation/1 -> Damping D1/1, omega_s/1  "d_omega"
  Accelerating power/1 -> Torque/1
  One/1 -> Speed deviation/2
  to own base/1 -> Accelerating power/2
  omega_s/1 -> Rotor angle/1
  Minus damping/1 -> 1 over 2H/1
  Rotor angle/1 -> delta [rad]/1  "delta"
  1 over 2H/1 -> Speed/1
  Speed/1 -> Speed deviation/1, Torque/2, omega [pu]/1  "omega"

== system case3_primary_AGC_GFM/SG1/Turbine (reheat) ==
  note: REHEAT STEAM TURBINE (IEEEG1, T7 = 0)
      | x_HP = gv/(1+sT4),  x_IP = x_HP/(1+sT5),  x_LP = x_IP/(1+sT6)
      | Pm = K1 x_HP + K3 x_IP + K5 x_LP
  valve gv [pu] : Inport
  Crossover T6 : Subsystem
      settings: AttributesFormatString=1/(1+s T6)
  HP fraction K1 : Gain  Gain=K1
  IP fraction K3 : Gain  Gain=K3
  LP fraction K5 : Gain  Gain=K5
  Reheater T5 : Subsystem
      settings: AttributesFormatString=1/(1+s T5)
  Steam chest T4 : Subsystem
      settings: AttributesFormatString=1/(1+s T4)
  Turbine power : Sum  Inputs=+++
  Pm [pu] : Outport
  wires:
  IP fraction K3/1 -> Turbine power/2
  Steam chest T4/1(x) -> HP fraction K1/1, Reheater T5/1(u)  "x_HP"
  valve gv [pu]/1 -> Steam chest T4/1(u)
  Turbine power/1 -> Pm [pu]/1  "Pm"
  LP fraction K5/1 -> Turbine power/3
  HP fraction K1/1 -> Turbine power/1
  Reheater T5/1(x) -> IP fraction K3/1, Crossover T6/1(u)  "x_IP"
  Crossover T6/1(x) -> LP fraction K5/1  "x_LP"

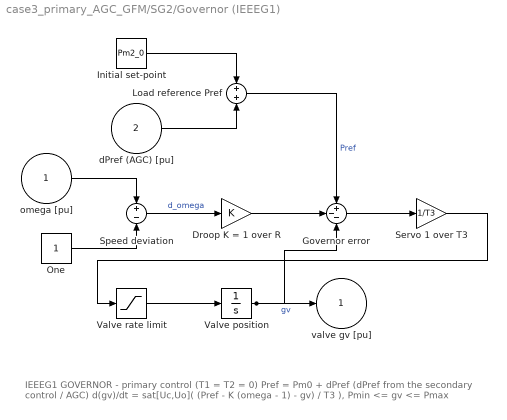
== system case3_primary_AGC_GFM/SG2/Governor (IEEEG1) ==
  note: IEEEG1 GOVERNOR - primary control (T1 = T2 = 0)
      | Pref = Pm0 + dPref   (dPref from the secondary control / AGC)
      | d(gv)/dt = sat[Uc,Uo]( (Pref - K (omega - 1) - gv) / T3 ),  Pmin <= gv <= Pmax
  omega [pu] : Inport
  dPref (AGC) [pu] : Inport  Port=2
  Droop K = 1 over R : Gain  Gain=K
  Governor error : Sum  Inputs=+--
  Initial set-point : Constant  Value=Pm2_0
  Load reference Pref : Sum
  One : Constant
  Servo 1 over T3 : Gain  Gain=1/T3
  Speed deviation : Sum  Inputs=+-
  Valve position : Integrator  InitialCondition=Pm2_0  LimitOutput=on  UpperSaturationLimit=Pmax  LowerSaturationLimit=Pmin
  Valve rate limit : Saturate  UpperLimit=Uo  LowerLimit=Uc
  valve gv [pu] : Outport
  wires:
  omega [pu]/1 -> Speed deviation/1
  Droop K = 1 over R/1 -> Governor error/2
  Load reference Pref/1 -> Governor error/1  "Pref"
  Speed deviation/1 -> Droop K = 1 over R/1  "d_omega"
  One/1 -> Speed deviation/2
  Initial set-point/1 -> Load reference Pref/1
  dPref (AGC) [pu]/1 -> Load reference Pref/2
  Valve rate limit/1 -> Valve position/1
  Valve position/1 -> Governor error/3, valve gv [pu]/1  "gv"
  Governor error/1 -> Servo 1 over T3/1
  Servo 1 over T3/1 -> Valve rate limit/1

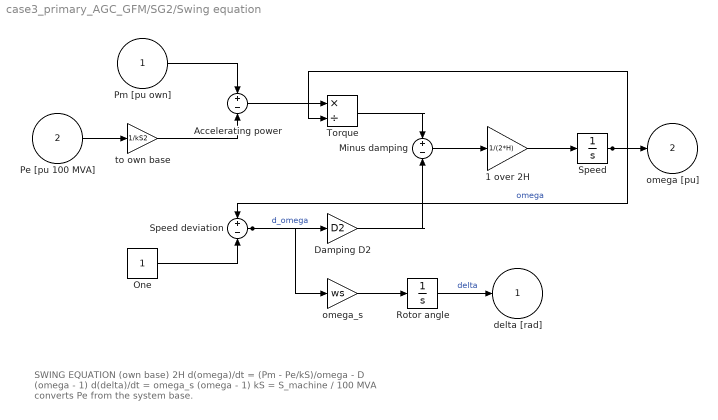
== system case3_primary_AGC_GFM/SG2/Swing equation ==
  note: SWING EQUATION (own base)
      | 2H d(omega)/dt = (Pm - Pe/kS)/omega - D (omega - 1)
      | d(delta)/dt    = omega_s (omega - 1)
      | kS = S_machine / 100 MVA converts Pe from the system base.
  Pm [pu own] : Inport
  Pe [pu 100 MVA] : Inport  Port=2
  1 over 2H : Gain  Gain=1/(2*H)
  Accelerating power : Sum  Inputs=+-
  Damping D2 : Gain  Gain=D2
  Minus damping : Sum  Inputs=+-
  One : Constant
  Rotor angle : Integrator  InitialCondition=delta2_0
  Speed : Integrator  InitialCondition=1
  Speed deviation : Sum  Inputs=+-
  Torque : Product  Inputs=*/
  omega_s : Gain  Gain=ws
  to own base : Gain  Gain=1/kS2
  delta [rad] : Outport
  omega [pu] : Outport  Port=2
  wires:
  Pe [pu 100 MVA]/1 -> to own base/1
  Damping D2/1 -> Minus damping/2
  Pm [pu own]/1 -> Accelerating power/1
  Torque/1 -> Minus damping/1
  Speed deviation/1 -> Damping D2/1, omega_s/1  "d_omega"
  Accelerating power/1 -> Torque/1
  One/1 -> Speed deviation/2
  to own base/1 -> Accelerating power/2
  omega_s/1 -> Rotor angle/1
  Minus damping/1 -> 1 over 2H/1
  Rotor angle/1 -> delta [rad]/1  "delta"
  1 over 2H/1 -> Speed/1
  Speed/1 -> Torque/2, Speed deviation/1, omega [pu]/1  "omega"

== system case3_primary_AGC_GFM/SG2/Turbine (reheat) ==
  note: REHEAT STEAM TURBINE (IEEEG1, T7 = 0)
      | x_HP = gv/(1+sT4),  x_IP = x_HP/(1+sT5),  x_LP = x_IP/(1+sT6)
      | Pm = K1 x_HP + K3 x_IP + K5 x_LP
  valve gv [pu] : Inport
  Crossover T6 : Subsystem
      settings: AttributesFormatString=1/(1+s T6)
  HP fraction K1 : Gain  Gain=K1
  IP fraction K3 : Gain  Gain=K3
  LP fraction K5 : Gain  Gain=K5
  Reheater T5 : Subsystem
      settings: AttributesFormatString=1/(1+s T5)
  Steam chest T4 : Subsystem
      settings: AttributesFormatString=1/(1+s T4)
  Turbine power : Sum  Inputs=+++
  Pm [pu] : Outport
  wires:
  valve gv [pu]/1 -> Steam chest T4/1(u)
  IP fraction K3/1 -> Turbine power/2
  Steam chest T4/1(x) -> HP fraction K1/1, Reheater T5/1(u)  "x_HP"
  Turbine power/1 -> Pm [pu]/1  "Pm"
  LP fraction K5/1 -> Turbine power/3
  HP fraction K1/1 -> Turbine power/1
  Reheater T5/1(x) -> IP fraction K3/1, Crossover T6/1(u)  "x_IP"
  Crossover T6/1(x) -> LP fraction K5/1  "x_LP"

== system case3_primary_AGC_GFM/Network/Source powers/SG1 power ==
  E : Inport
  V : Inport  Port=2
  1 over jxd1 : Gain  Gain=1/(1i*xd1)
  E - V : Sum  Inputs=+-
  P and Q : ComplexToRealImag
  S : Product
  conj I : Math  Operator=conj
  Pe : Outport
  Qe : Outport  Port=2
  wires:
  E - V/1 -> 1 over jxd1/1
  E/1 -> E - V/1
  P and Q/1 -> Pe/1
  V/1 -> E - V/2, S/1
  1 over jxd1/1 -> conj I/1  "I"
  P and Q/2 -> Qe/1
  S/1 -> P and Q/1
  conj I/1 -> S/2

== system case3_primary_AGC_GFM/Network/Source powers/SG2 power ==
  E : Inport
  V : Inport  Port=2
  1 over jxd2 : Gain  Gain=1/(1i*xd2)
  E - V : Sum  Inputs=+-
  P and Q : ComplexToRealImag
  S : Product
  conj I : Math  Operator=conj
  Pe : Outport
  Qe : Outport  Port=2
  wires:
  E/1 -> E - V/1
  V/1 -> E - V/2, S/1
  E - V/1 -> 1 over jxd2/1
  1 over jxd2/1 -> conj I/1  "I"
  P and Q/2 -> Qe/1
  S/1 -> P and Q/1
  conj I/1 -> S/2
  P and Q/1 -> Pe/1

== system case3_primary_AGC_GFM/SG1/Turbine (reheat)/Crossover T6 ==
  u : Inport
  Error : Sum  Inputs=+-
  One over T : Gain  Gain=1/T6
  State : Integrator  InitialCondition=Pm1_0
  x : Outport
  wires:
  State/1 -> Error/2, x/1
  u/1 -> Error/1
  Error/1 -> One over T/1
  One over T/1 -> State/1

== system case3_primary_AGC_GFM/SG1/Turbine (reheat)/Reheater T5 ==
  u : Inport
  Error : Sum  Inputs=+-
  One over T : Gain  Gain=1/T5
  State : Integrator  InitialCondition=Pm1_0
  x : Outport
  wires:
  State/1 -> Error/2, x/1
  u/1 -> Error/1
  Error/1 -> One over T/1
  One over T/1 -> State/1

== system case3_primary_AGC_GFM/SG1/Turbine (reheat)/Steam chest T4 ==
  u : Inport
  Error : Sum  Inputs=+-
  One over T : Gain  Gain=1/T4
  State : Integrator  InitialCondition=Pm1_0
  x : Outport
  wires:
  One over T/1 -> State/1
  u/1 -> Error/1
  State/1 -> x/1, Error/2
  Error/1 -> One over T/1

== system case3_primary_AGC_GFM/SG2/Turbine (reheat)/Crossover T6 ==
  u : Inport
  Error : Sum  Inputs=+-
  One over T : Gain  Gain=1/T6
  State : Integrator  InitialCondition=Pm2_0
  x : Outport
  wires:
  State/1 -> Error/2, x/1
  u/1 -> Error/1
  Error/1 -> One over T/1
  One over T/1 -> State/1

== system case3_primary_AGC_GFM/SG2/Turbine (reheat)/Reheater T5 ==
  u : Inport
  Error : Sum  Inputs=+-
  One over T : Gain  Gain=1/T5
  State : Integrator  InitialCondition=Pm2_0
  x : Outport
  wires:
  State/1 -> Error/2, x/1
  u/1 -> Error/1
  Error/1 -> One over T/1
  One over T/1 -> State/1

== system case3_primary_AGC_GFM/SG2/Turbine (reheat)/Steam chest T4 ==
  u : Inport
  Error : Sum  Inputs=+-
  One over T : Gain  Gain=1/T4
  State : Integrator  InitialCondition=Pm2_0
  x : Outport
  wires:
  One over T/1 -> State/1
  u/1 -> Error/1
  State/1 -> Error/2, x/1
  Error/1 -> One over T/1
